simulink model "BatterySystemSOC_AI"  (R2026b)
settings: Solver=FixedStepAuto
model workspace (MAT data in the model file):
  systemNetwork = dlnetwork
  systemNetwork.any.Version = 7
  systemNetwork.any.LayerGraph = nnet.cnn.LayerGraph
  systemNetwork.any.LayerGraph.any.Version = 1
  systemNetwork.any.LayerGraph.any.Layers(1) = nnet.cnn.layer.FeatureInputLayer
  systemNetwork.any.LayerGraph.any.Layers(1).any.Version = 2
  systemNetwork.any.LayerGraph.any.Layers(1).any.Name = 'input'
  systemNetwork.any.LayerGraph.any.Layers(1).any.InputSize = 3
  systemNetwork.any.LayerGraph.any.Layers(1).any.Normalization.Version = 1
  systemNetwork.any.LayerGraph.any.Layers(1).any.Normalization.Type = 'zscore'
  systemNetwork.any.LayerGraph.any.Layers(1).any.Normalization.ImageSize = 3
  systemNetwork.any.LayerGraph.any.Layers(1).any.Normalization.Mean = [3.51086234612; 1.90519027601; 29.8811166481]
  systemNetwork.any.LayerGraph.any.Layers(1).any.Normalization.Std = [0.32451522033; 1.13732968399; 8.63659704385]
  systemNetwork.any.LayerGraph.any.Layers(1).any.NormalizationDimension = 'auto'
  systemNetwork.any.LayerGraph.any.Layers(1).any.SplitComplexInputs = 0
  systemNetwork.any.LayerGraph.any.Layers(2) = nnet.cnn.layer.FullyConnectedLayer
  systemNetwork.any.LayerGraph.any.Layers(2).any.Version = 5
  systemNetwork.any.LayerGraph.any.Layers(2).any.Name = 'fc_1'
  systemNetwork.any.LayerGraph.any.Layers(2).any.InputSize = []
  systemNetwork.any.LayerGraph.any.Layers(2).any.OutputSize = 12
  systemNetwork.any.LayerGraph.any.Layers(2).any.Weights.Version = 2
  systemNetwork.any.LayerGraph.any.Layers(2).any.Weights.Value = [-0.357126653194  -0.167446419597  0.313396573067; 0.133876234293  -0.372911691666  -0.327937602997; 0.0143512431532  -0.207290768623  -0.131954982877; -0.0940770059824  0.436393916607  0.231666103005; 0.572077035904  -0.10127235204  0.0312585830688; -0.0145770041272  -0.0032209395431  0.00279129017144; 0.222840875387  0.344052165747  -0.288534730673; -0.632789492607  -0.315690755844  0.031650826335; -0.41238284111  0.0755508467555  -0.0226038098335; 0.493653208017  0.200725868344  -0.00207745656371; 0.12494212389  -0.236405938864  -0.107543773949; 0.378771930933  0.223037242889  -0.0354217514396]
  systemNetwork.any.LayerGraph.any.Layers(2).any.Weights.LearnRateFactor = 1
  systemNetwork.any.LayerGraph.any.Layers(2).any.Weights.L2Factor = 1
  systemNetwork.any.LayerGraph.any.Layers(2).any.Weights.Initializer.Version = 1
  systemNetwork.any.LayerGraph.any.Layers(2).any.Weights.Initializer.Class = 'nnet.internal.cnn.layer.learnable.initializer.Glorot'
  systemNetwork.any.LayerGraph.any.Layers(2).any.Weights.Initializer.ConstructorArguments = {2, 1}
  systemNetwork.any.LayerGraph.any.Layers(2).any.Bias.Version = 2
  systemNetwork.any.LayerGraph.any.Layers(2).any.Bias.Value = [-0.0487607456744; -0.0485792607069; 0.0573302358389; 0.0139646762982; 0.0598504394293; -0.0895017758012; 0.0728969275951; -0.0860656574368; -0.0316937975585; 0.0937769412994; -0.0544996112585; 0.0210902541876]
  systemNetwork.any.LayerGraph.any.Layers(2).any.Bias.LearnRateFactor = 1
  systemNetwork.any.LayerGraph.any.Layers(2).any.Bias.L2Factor = 0
  systemNetwork.any.LayerGraph.any.Layers(2).any.Bias.Initializer.Version = 1
  systemNetwork.any.LayerGraph.any.Layers(2).any.Bias.Initializer.Class = 'nnet.internal.cnn.layer.learnable.initializer.Zeros'
  systemNetwork.any.LayerGraph.any.Layers(2).any.Bias.Initializer.ConstructorArguments = []
  systemNetwork.any.LayerGraph.any.Layers(2).any.InputLearnables = {}
  systemNetwork.any.LayerGraph.any.Layers(2).any.OutputLearnables = {}
  systemNetwork.any.LayerGraph.any.Layers(2).any.OperationDimension = 'spatial-channel'
  systemNetwork.any.LayerGraph.any.Layers(3) = nnet.cnn.layer.ReLULayer
  systemNetwork.any.LayerGraph.any.Layers(3).any.Version = 1
  systemNetwork.any.LayerGraph.any.Layers(3).any.Name = 'relu'
  systemNetwork.any.LayerGraph.any.Layers(4) = nnet.cnn.layer.FullyConnectedLayer
  systemNetwork.any.LayerGraph.any.Layers(4).any.Version = 5
  systemNetwork.any.LayerGraph.any.Layers(4).any.Name = 'fc_2'
  systemNetwork.any.LayerGraph.any.Layers(4).any.InputSize = []
  systemNetwork.any.LayerGraph.any.Layers(4).any.OutputSize = 1
  systemNetwork.any.LayerGraph.any.Layers(4).any.Weights.Version = 2
  systemNetwork.any.LayerGraph.any.Layers(4).any.Weights.Value = [-0.00755796395242 0.00673354044557 0.0470778010786 -0.0378492772579 0.165892228484 -0.127779096365 0.00474803894758 -0.257535904646 -0.237768501043 0.199417442083 0.0221268124878 0.190935313702]
  systemNetwork.any.LayerGraph.any.Layers(4).any.Weights.LearnRateFactor = 1
  systemNetwork.any.LayerGraph.any.Layers(4).any.Weights.L2Factor = 1
  systemNetwork.any.LayerGraph.any.Layers(4).any.Weights.Initializer.Version = 1
  systemNetwork.any.LayerGraph.any.Layers(4).any.Weights.Initializer.Class = 'nnet.internal.cnn.layer.learnable.initializer.Glorot'
  systemNetwork.any.LayerGraph.any.Layers(4).any.Weights.Initializer.ConstructorArguments = {2, 1}
  systemNetwork.any.LayerGraph.any.Layers(4).any.Bias.Version = 2
  systemNetwork.any.LayerGraph.any.Layers(4).any.Bias.Value = 0.461965799332
  systemNetwork.any.LayerGraph.any.Layers(4).any.Bias.LearnRateFactor = 1
  systemNetwork.any.LayerGraph.any.Layers(4).any.Bias.L2Factor = 0
  systemNetwork.any.LayerGraph.any.Layers(4).any.Bias.Initializer.Version = 1
  systemNetwork.any.LayerGraph.any.Layers(4).any.Bias.Initializer.Class = 'nnet.internal.cnn.layer.learnable.initializer.Zeros'
  systemNetwork.any.LayerGraph.any.Layers(4).any.Bias.Initializer.ConstructorArguments = []
  systemNetwork.any.LayerGraph.any.Layers(4).any.InputLearnables = {}
  systemNetwork.any.LayerGraph.any.Layers(4).any.OutputLearnables = {}
  systemNetwork.any.LayerGraph.any.Layers(4).any.OperationDimension = 'spatial-channel'
  systemNetwork.any.LayerGraph.any.Connections = table
  systemNetwork.any.LayerGraph.any.Connections.data = {{'input'; 'fc_1'; 'relu'}, {'fc_1'; 'relu'; 'fc_2'}}
  systemNetwork.any.LayerGraph.any.Connections.ndims = 2
  systemNetwork.any.LayerGraph.any.Connections.nrows = 3
  systemNetwork.any.LayerGraph.any.Connections.nvars = 2
  systemNetwork.any.LayerGraph.any.Connections.varnames = {'Source', 'Destination'}
  systemNetwork.any.LayerGraph.any.Connections.props.CustomProps = struct()
  systemNetwork.any.LayerGraph.any.Connections.props.VariableCustomProps = struct()
  systemNetwork.any.LayerGraph.any.Connections.props.versionSavedFrom = 5
  systemNetwork.any.LayerGraph.any.Connections.props.minCompatibleVersion = 1
  systemNetwork.any.LayerGraph.any.Connections.props.incompatibilityMsg = ''
  systemNetwork.any.LayerGraph.any.Connections.props.VersionSavedFrom = 5
  systemNetwork.any.LayerGraph.any.Connections.props.useVariableNamesOriginal = 0
  systemNetwork.any.LayerGraph.any.Connections.props.useVariableNames2048 = 0
  systemNetwork.any.LayerGraph.any.Connections.props.useDimensionNamesOriginal = 0
  systemNetwork.any.LayerGraph.any.Connections.props.useDimensionNames2048 = 0
  systemNetwork.any.LayerGraph.any.Connections.props.Description = ''
  systemNetwork.any.LayerGraph.any.Connections.props.VariableNamesOriginal = {}
  systemNetwork.any.LayerGraph.any.Connections.props.VariableNames2048 = {}
  systemNetwork.any.LayerGraph.any.Connections.props.DimensionNames = {'Row', 'Variables'}
  systemNetwork.any.LayerGraph.any.Connections.props.DimensionNamesOriginal = {}
  systemNetwork.any.LayerGraph.any.Connections.props.DimensionNames2048 = {}
  systemNetwork.any.LayerGraph.any.Connections.props.UserData = []
  systemNetwork.any.LayerGraph.any.Connections.props.VariableDescriptions = {}
  systemNetwork.any.LayerGraph.any.Connections.props.VariableUnits = {}
  systemNetwork.any.LayerGraph.any.Connections.props.VariableContinuity = {}
  systemNetwork.any.Initialized = 1
  systemNetwork.any.SerializedQuantizationInfo.version = 1
  systemNetwork.any.SerializedQuantizationInfo.data = containers.Map
  systemNetwork.any.SerializedQuantizationInfo.data.serialization.keys = {}
  systemNetwork.any.SerializedQuantizationInfo.data.serialization.values = {}
  systemNetwork.any.SerializedQuantizationInfo.data.serialization.uniformity = 0
  systemNetwork.any.SerializedQuantizationInfo.data.serialization.keyType = 'char'
  systemNetwork.any.SerializedQuantizationInfo.data.serialization.valueType = 'any'
  systemNetwork.any.ExampleInputs = {}
  systemNetwork.any.OutputNames = {'fc_2'}
  systemNetwork.any.ExternalOutputNames = []
  systemNetwork.any.ExternalInputNames = []
  systemNetwork.any.RetainCustomInputNames = 1
  systemNetwork.any.RetainCustomOutputNames = 1
  systemNetwork.any.InitializationMode = "size"
libraries: dlconvfclib x2, dlinputlayernormlib x1, dlactivationlib x1
settings Model: Creator=mgado  LastModifiedBy=mgado
settings OptimizationCC: DefaultParameterBehavior=Inlined  DifferentSizesBufferReuse=on  EfficientTunableParamExpr=on  EnhancedBackFolding=on  OptimizationCustomize=off  OptimizeBlockOrder=speed  PassReuseOutputArgsAs=Individual arguments  RemoveInternalMemoryZeroInit=on  RemoveRootLevelIOMemoryZeroInit=on
settings DebuggingCC: ParameterTunabilityLossMsg=error
settings SFSimCC: MATLABDynamicMemAlloc=off
settings RTWCC: DataTypeReplacement=CDataTypesFixedWidth  Description=Embedded Coder  SystemTargetFile=ert.tlc  TemplateMakefile=ert_default_tmf
settings CodeAppCC: ForceParamTrailComments=on  IgnoreCustomStorageClasses=off  InsertBlockDesc=on  OperatorAnnotations=on  SFDataObjDesc=on  SimulinkDataObjDesc=on
settings ERTTargetCC: CombineSignalStateStructs=on  GenerateSampleERTMain=on  MaxIdInt16=INT16_MAX  MaxIdInt32=INT32_MAX  MaxIdInt64=INT64_MAX  MaxIdInt8=INT8_MAX  MaxIdUint16=UINT16_MAX  MaxIdUint32=UINT32_MAX  MaxIdUint64=UINT64_MAX  MaxIdUint8=UINT8_MAX  MinIdInt16=INT16_MIN  MinIdInt32=INT32_MIN  MinIdInt64=INT64_MIN  MinIdInt8=INT8_MIN

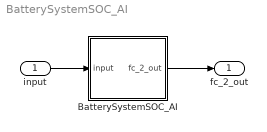
== system BatterySystemSOC_AI ==
  input : Inport  PortDimensions=[3]  SampleTime=1
  BatterySystemSOC_AI : Subsystem
  fc_2_out : Outport
  wires:
  input/1 -> BatterySystemSOC_AI/1(input)
  BatterySystemSOC_AI/1(fc_2_out) -> fc_2_out/1

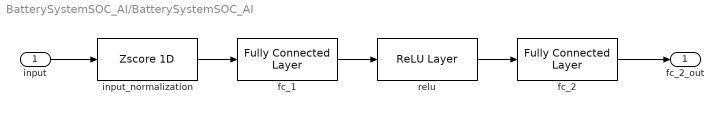
== system BatterySystemSOC_AI/BatterySystemSOC_AI ==
  input : Inport  PortDimensions=[3]  SampleTime=1
  fc_1 : dlconvfclib/Fully Connected Layer  Layer=systemNetwork.Layers(2)  InputSize=1  OutMin=[]  OutMax=[]  WeightsDataTypeStr=Inherit: Inherit via back propagation  WeightsMin=[]  WeightsMax=[]  BiasDataTypeStr=Inherit: Inherit via back propagation  BiasMin=[]  BiasMax=[]  AccumMin=[]  AccumMax=[]  InternalRndMeth=Floor  InternalSaturateOnIntegerOverflow=off  SampleTime=1
      settings: DataFormat=C
  fc_2 : dlconvfclib/Fully Connected Layer  Layer=systemNetwork.Layers(4)  InputSize=1  OutMin=[]  OutMax=[]  WeightsDataTypeStr=Inherit: Inherit via back propagation  WeightsMin=[]  WeightsMax=[]  BiasDataTypeStr=Inherit: Inherit via back propagation  BiasMin=[]  BiasMax=[]  AccumMin=[]  AccumMax=[]  InternalRndMeth=Floor  InternalSaturateOnIntegerOverflow=off  SampleTime=1
      settings: DataFormat=C
  input_normalization : dlinputlayernormlib/Zscore 1D  Layer=systemNetwork.Layers(1)  OutMin=[]  OutMax=[]  MeanDataTypeStr=Inherit: Inherit via back propagation  MeanMin=[]  MeanMax=[]  StandardDeviationDataTypeStr=Inherit: Inherit via back propagation  StandardDeviationMin=[]  StandardDeviationMax=[]  AccumMin=[]  AccumMax=[]  InternalRndMeth=Floor  InternalSaturateOnIntegerOverflow=off  SampleTime=1
      settings: DataFormat=C
  relu : dlactivationlib/ReLU Layer  OutMin=[]  OutMax=[]  SampleTime=1
  fc_2_out : Outport
  wires:
  input/1 -> input_normalization/1
  input_normalization/1 -> fc_1/1
  fc_1/1 -> relu/1
  relu/1 -> fc_2/1
  fc_2/1 -> fc_2_out/1
